simulink model "FOC_physical_2"  (R2024b)
settings: Solver=FixedStepAuto  StartTime=0.0  StopTime=3  FixedStep=1e-5  RelTol=1e-3
undefined symbols (not defined in the file): Down, GPTRIP1SEL, Ki_current, Ki_q, Ki_s, Ki_speed, Kp_current, Kp_q, Kp_s, Kp_speed, lambda, lamdaM, Ld, Ls, ma, P, Rs, T_max, T_period, Ts, TZ1, Up, Vdc
libraries: simulink x8, spsIGBTDiodeLib x6, spsCurrentMeasurementLib x3, eeStairGenerator x3, nesl_utility x2, spsDCVoltageSourceLib x1, spsPermanentMagnetSynchronousMachineLib x1, c2802xlib x1, spsThreePhaseVIMeasurementLib x1, spsVoltageMeasurementLib x1, sps_lib x1
(part 1 of 2)
settings Model: Creator=ahmed  LastModifiedBy=ahmed
settings SolverCC: ZeroCrossAlgorithm=Adaptive
settings DebuggingCC: IgnoredZcDiagnostic=none

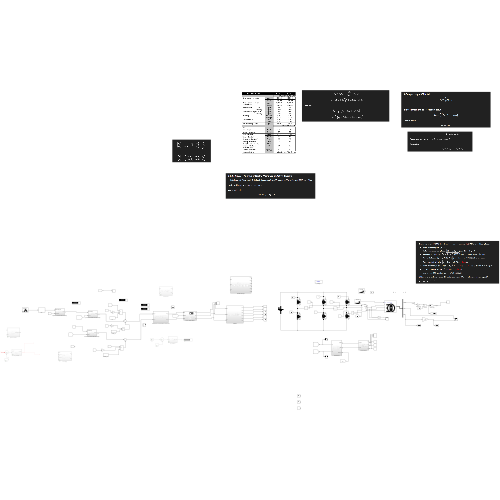
[thumbnail: Simulink's stored preview of the top-level diagram]
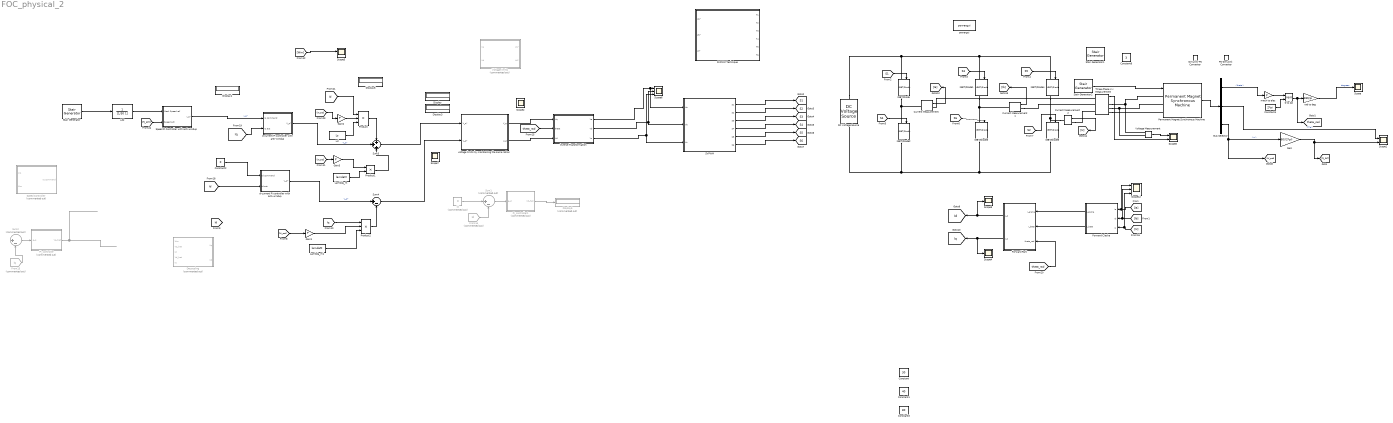
== system FOC_physical_2 ==
  0 to 2pi : Math  Operator=rem
  Bus Selector : BusSelector  OutputSignals=theta,Te,w
  Constant : Constant  Value=30
  Constant1 : Constant  Value=40
  Constant2 : Constant  Value=0
  Constant3 : Constant  Value=80
  Constant4 : Constant  Value=2*pi
  Constant6 : Constant  Value=3
  Current Measurement : spsCurrentMeasurementLib/Current Measurement  PhasorSimulation=off  OutputType=Complex  PSBequivalent=0
  Current Measurement1 : spsCurrentMeasurementLib/Current Measurement  PhasorSimulation=off  OutputType=Complex  PSBequivalent=0
  Current Measurement2 : spsCurrentMeasurementLib/Current Measurement  PhasorSimulation=off  OutputType=Complex  PSBequivalent=0
  DC Voltage Source : spsDCVoltageSourceLib/DC Voltage Source  Amplitude=Vdc  Measurements=None
  "Decoupling " : Subsystem  Commented=on
  Display{,3..4,6} (4 alike) : Display
  Display5 : Display  Commented=on
  Forward Clacke : Subsystem
  Forward Park : Subsystem
  From13 : From  Commented=on  GotoTag=Iq  TagVisibility=global
  From14 : From  Commented=on  GotoTag=Id  TagVisibility=global
  Gain : Gain  Gain=60/(2*pi)
  Gain1 : Gain  Gain=P
  Gain2 : Gain  Gain=P
  Gain3 : Gain  Gain=P
  IGBT/Diode{,1..5} (6 alike) : spsIGBTDiodeLib/IGBT//Diode  Ron=1e-3  Rs=1e5  Cs=inf  Measurements=on
  Id : Constant  Commented=on  Value=0
  Inverse Transformation : Subsystem
  LPF : TransferFcn  Denominator=[1/30 1]
  Lambda_m : Constant  Value=lamdaM
  Lambda_m1 : Constant  Value=lamdaM
  Ld : Constant  Value=Ls
  PI_controller : Subsystem  Commented=on
  PI_controller1 : Subsystem  Commented=on
  PS-Simulink Converter : nesl_utility/PS-Simulink Converter  PhysicalDomain=network_engine_domain  SubClassName=ps_output  LeftPortType=input  RightPortType=output  PseudoPeriodic=off  Frequencies=[]  VectorFormat=inherit  Unit=inherit  AffineConversion=off
  Permanent Magnet Synchronous Machine : spsPermanentMagnetSynchronousMachineLib/Permanent Magnet Synchronous Machine  NbPhases=3  FluxDistribution=Sinusoidal  RotorType=Round  MechanicalLoad=Torque Tm  PresetModel=No  ShowDetailedParameters=on  MeasurementBus=on  Resistance=Rs  Inductance=8.5e-3  dqInductances=[6.2e-3 6.2e-3]  La=Ls  MachineConstant=Flux linkage established by magnets (V.s)  Flux=.0620  VoltageCst=44.9822  TorqueCst=0.372  Flat=120  Mechanical=[2.6e-5 9.55e-5 4 .03]  PolePairs=4  InitialConditions=[0,0, 0,0]  InitialConditions5ph=[0 0 0 0 0 0]  RefAngle=Aligned with phase A axis (original Park)  IterativeDiscreteModel=Trapezoidal non iterative  TsBlock=-1  TsPowergui=0
  Product : Product  Inputs=3
  Product1 : Product
  Product2 : Product  Inputs=3
  SVPWM : Subsystem
  SVPWM Technique : Subsystem
  Scope : Scope
  Scope1 : Scope  NumInputPorts=2
  Scope{2,6..7,12} (4 alike) : Scope  NumInputPorts=3
  Scope3 : Scope
  Scope4 : Scope
  Scope5 : Scope  NumInputPorts=2
  Scope8 : Scope  NumInputPorts=2
  Simulink-PS Converter : nesl_utility/Simulink-PS Converter  PhysicalDomain=network_engine_domain  SubClassName=ps_input  LeftPortType=input  RightPortType=output  PseudoPeriodic=off  Frequencies=[]  NoiseDistribution=none  NoiseParameters=[]  Unit=1  AffineConversion=off  FilteringAndDerivatives=provide  SimscapeFilterOrder=1  InputFilterTimeConstant=0.001  UdotUserProvided=0
  "Speed Controller " : Subsystem  Commented=on
  Speed PI Controller with anti-windup : Subsystem
  Stair Generator : eeStairGenerator/Stair Generator  LabelModeActiveChoice=Discrete  TimeInput=[0.2 .6 1 1.3 1.8 2.2 3]  AmplitudeInput=[200 300 1000 4000 4500 2000 0]  SampleTime=1e-5  RepeatPattern=off  OutDataTypeStr=double
      settings: LibrarySourceBlock=ee_sl_lib/General Control/Stair Generator
  Stair Generator1 : eeStairGenerator/Stair Generator  LabelModeActiveChoice=Discrete  TimeInput=[0.3 .6 1.2 1.8]  AmplitudeInput=[.5 1 1.2 3]  SampleTime=Ts  RepeatPattern=off  OutDataTypeStr=double
      settings: LibrarySourceBlock=ee_sl_lib/General Control/Stair Generator
  Stair Generator2 : eeStairGenerator/Stair Generator  LabelModeActiveChoice=Discrete  TimeInput=[0.3 .7]  AmplitudeInput=[.6 1]  SampleTime=1e-5  RepeatPattern=off  OutDataTypeStr=double
      settings: LibrarySourceBlock=ee_sl_lib/General Control/Stair Generator
  Sum1 : Sum  Commented=on  Inputs=|+-
  Sum2 : Sum  Commented=on  Inputs=|+-
  Sum3 : Sum  Inputs=+++
  Sum4 : Sum  Inputs=|+-
  Three-Phase V-I Measurement : spsThreePhaseVIMeasurementLib/Three-Phase V-I Measurement  VoltageMeasurement=phase-to-ground  SetLabelV=off  LabelV=Vabc  Vpu=off  VpuLL=off  CurrentMeasurement=yes  SetLabelI=off  LabelI=Iabc  Ipu=off  Pbase=100e6  Vbase=500e3  OutputType=Complex  PhasorSimulation=off  PSBequivalent=0
  Voltage Measurement : spsVoltageMeasurementLib/Voltage Measurement  PhasorSimulation=off  OutputType=Complex  PSBequivalent=0
  Voltage limits : Subsystem  Commented=on
  d-current PI controller with anti-windup : Subsystem
  mech to elec : Gain  Gain=P
  powergui : sps_lib/powergui  Priority=1  SimulationMode=Discrete  SampleTime=1e-5  frequency=60  Iterations=50  frequencyindice=0  Pbase=100e6  ErrMax=1e-4  UnitsV=kV  UnitsW=MW  buscounter=0  FunctionMessages=off  echomessages=off  EnableUseOfTLC=off  CurrentSourceSwitches=off  DisableSnubberDevices=off  DisableRonSwitches=off  DisableVfSwitches=off  DisplayEquations=off  AutomaticDiscreteSolvers=off  SolverType=Tustin/Backward Euler (TBE)  Interpol=off  ExternalGateDelay=off  methode=off  Ts=100  x0status=blocks  SPID=on  SwTol=0  HookPort=off  NonlinearTolerance=1e-4  nMaxIteration=100  ContinueOnMaxIteration=off  RestoreLinks=warning  ResistiveCurrentMeasurement=off  Frange=[0:2:500]  Ylog=off  Xlog=on  ShowGrid=off  save=off  variable=ZData  structure=0  ZoomFFT=off  StartTime=0.0  cycles=1  DisplayStyle=1  fundamental=60  FreqAxis=off  MaxFrequency=1000  frequencyindicesteady=1  RmsSteady=1  display=off
  q-current PI controller with anti-windup : Subsystem
  rad to deg : Gain  Gain=180/pi
  voltage limits by maintaining the same ration : Subsystem
  tag scope: Id=global, Iq=global, S1=global, S2=global, S3=global, S4=global, S5=global, S6=global, theta_rad=global
  wires:
  Permanent Magnet Synchronous Machine/1 -> Bus Selector/1
  [S3] -> IGBT/Diode1/1
  [S6] -> IGBT/Diode3/1
  [S5] -> IGBT/Diode4/1
  [S4] -> IGBT/Diode2/1
  [S1] -> IGBT/Diode/1
  [S2] -> IGBT/Diode5/1
  [Wm] -> Scope5/1
  PI_controller1/1(Vd_hat) -> Display5/1
  Id/1 -> Sum1/1
  Inverse Transformation/1(Va) -> SVPWM/1(Va), Scope6/1
  Inverse Transformation/3(Vc) -> SVPWM/3(Vc), Scope6/3
  [theta_rad] -> Inverse Transformation/2(theta)
  Inverse Transformation/2(Vb) -> SVPWM/2(Vb), Scope6/2
  From14/1 -> Sum1/2
  [Ic] -> Forward Clacke/3(Ic), Scope12/3
  [Ia] -> Forward Clacke/1(Ia), Scope12/1
  Forward Clacke/2(I_beta) -> Forward Park/2(I_beta)
  [Ib] -> Forward Clacke/2(Ib), Scope12/2
  Forward Clacke/1(I_alpha) -> Forward Park/1(I_alpha)
  Forward Park/1(I_d) -> [Id], Scope3/1
  Forward Park/2(I_q) -> [Iq], Scope4/1
  Current Measurement/1 -> [Ia]
  Current Measurement1/1 -> [Ib]
  voltage limits by maintaining the same ration/1(V_q) -> Inverse Transformation/1(Vq)
  voltage limits by maintaining the same ration/2(V_d) -> Inverse Transformation/3(Vd)
  Sum1/1 -> PI_controller1/1(e_d)
  Constant2/1 -> d-current PI controller with anti-windup/1(Id command)
  [Id] -> d-current PI controller with anti-windup/2(Id act)
  ? -> Sum2/1
  Sum2/1 -> PI_controller/1(e_q)
  PI_controller/1(Vq_hat) -> ?
  From13/1 -> Sum2/2
  [Iq] -> q-current PI controller with anti-windup/2(Iq act)
  LPF/1 -> Speed PI Controller with anti-windup/1(Mech Speed ref)
  Speed PI Controller with anti-windup/1(I_q*) -> q-current PI controller with anti-windup/1(Iq command)  "I_q*"
  Product/1 -> Sum3/1
  [Iq] -> Product2/1
  Product1/1 -> Sum3/3
  Lambda_m1/1 -> Product2/3
  Lambda_m/1 -> Product1/2
  Ld/1 -> Product/3
  [W_act] -> Gain3/1
  Product2/1 -> Sum4/2
  [Id] -> Product/1
  q-current PI controller with anti-windup/1(V_q*) -> Sum3/2  "V_q*"
  Sum3/1 -> voltage limits by maintaining the same ration/1(V_q*)
  d-current PI controller with anti-windup/1(V_d*) -> Sum4/1  "V_d*"
  Sum4/1 -> voltage limits by maintaining the same ration/2(V_d*)
  Bus Selector/2 -> Scope1/1  "<Te>"
  Bus Selector/3 -> Gain/1, [W_act]  "<w>"
  Bus Selector/1 -> mech to elec/1  "<theta>"
  0 to 2pi/1 -> rad to deg/1, [theta_rad]
  Constant4/1 -> 0 to 2pi/2
  rad to deg/1 -> Scope/1  "degrees"
  mech to elec/1 -> 0 to 2pi/1
  Gain/1 -> Scope1/2, [N_act]
  [N_act] -> Speed PI Controller with anti-windup/2(Speed act)
  [W_act] -> Gain1/1
  [theta_rad] -> Forward Park/3(theta_rad)
  Current Measurement2/1 -> [Ic]
  Gain1/1 -> Product2/2
  [W_act] -> Gain2/1
  Gain2/1 -> Product/2
  SVPWM/1(S1) -> [S1]
  SVPWM/2(S2) -> [S2]
  SVPWM/3(S3) -> [S3]
  SVPWM/4(S4) -> [S4]
  SVPWM/5(S5) -> [S5]
  SVPWM/6(S6) -> [S6]
  Stair Generator/1 -> LPF/1
  Stair Generator2/1 -> Permanent Magnet Synchronous Machine/1
  Gain3/1 -> Product1/1
  Voltage Measurement/1 -> Scope8/1
  Three-Phase V-I Measurement/1 -> Scope8/2
  connections:
  DC Voltage Source/RConn1 -- IGBT/Diode4/LConn1 -- IGBT/Diode1/LConn1 -- IGBT/Diode/LConn1
  Current Measurement/LConn1 -- IGBT/Diode/RConn1 -- IGBT/Diode2/LConn1
  Current Measurement2/LConn1 -- IGBT/Diode4/RConn1 -- IGBT/Diode5/LConn1
  DC Voltage Source/LConn1 -- IGBT/Diode5/RConn1 -- IGBT/Diode3/RConn1 -- IGBT/Diode2/RConn1
  Current Measurement1/LConn1 -- IGBT/Diode1/RConn1 -- IGBT/Diode3/LConn1
  Voltage Measurement/LConn1 -- Permanent Magnet Synchronous Machine/LConn1 -- Three-Phase V-I Measurement/RConn1
  Voltage Measurement/LConn2 -- Permanent Magnet Synchronous Machine/LConn2 -- Three-Phase V-I Measurement/RConn2
  Current Measurement2/RConn1 -- Three-Phase V-I Measurement/LConn3
  Current Measurement1/RConn1 -- Three-Phase V-I Measurement/LConn2
  Three-Phase V-I Measurement/LConn1 -- Current Measurement/RConn1
  Three-Phase V-I Measurement/RConn3 -- Permanent Magnet Synchronous Machine/LConn3

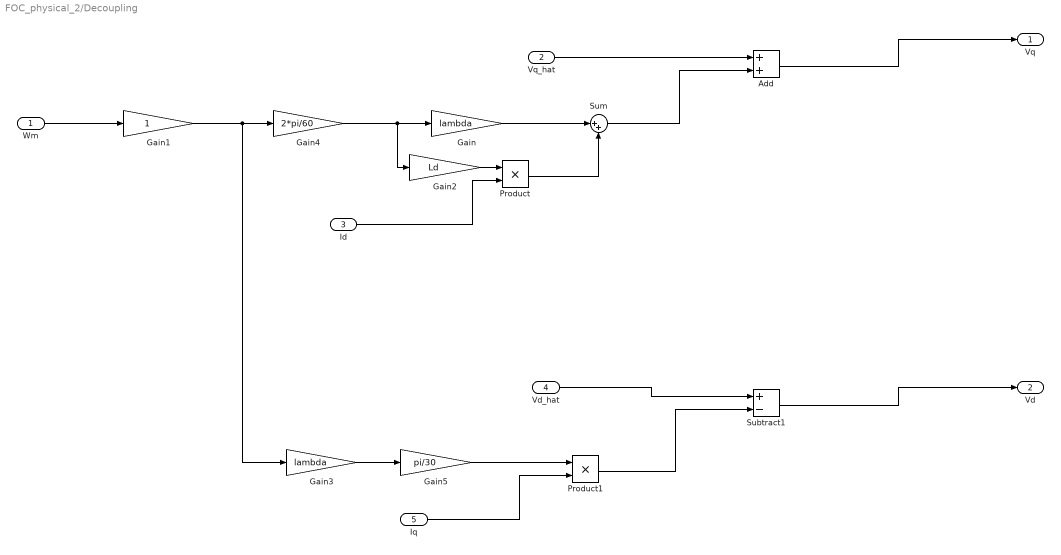
== system FOC_physical_2/Decoupling  ==
  Wm : Inport
  Vq_hat : Inport  Port=2
  Id : Inport  Port=3
  Vd_hat : Inport  Port=4
  Iq : Inport  Port=5
  Add : Sum
  Gain : Gain  Gain=lambda
  Gain1 : Gain
  Gain2 : Gain  Gain=Ld
  Gain3 : Gain  Gain=lambda
  Gain4 : Gain  Gain=2*pi/60
  Gain5 : Gain  Gain=pi/30
  Product : Product
  Product1 : Product
  Subtract1 : Sum  Inputs=+-
  Sum : Sum  Inputs=|++
  Vq : Outport
  Vd : Outport  Port=2
  wires:
  Vq_hat/1 -> Add/1
  Vd_hat/1 -> Subtract1/1
  Wm/1 -> Gain1/1
  Gain1/1 -> Gain4/1, Gain3/1
  Gain2/1 -> Product/1
  Id/1 -> Product/2
  Product/1 -> Sum/2
  Gain/1 -> Sum/1
  Sum/1 -> Add/2
  Gain3/1 -> Gain5/1
  Product1/1 -> Subtract1/2
  Iq/1 -> Product1/2
  Gain4/1 -> Gain2/1, Gain/1
  Add/1 -> Vq/1
  Subtract1/1 -> Vd/1
  Gain5/1 -> Product1/1

== system FOC_physical_2/Forward Clacke ==
  Ia : Inport
  Ib : Inport  Port=2
  Ic : Inport  Port=3
  Gain : Gain  Gain=0.5
  Gain1 : Gain  Gain=0.5
  Gain2 : Gain  Gain=2/3
  Gain3 : Gain  Gain=sqrt(3)/2
  Gain4 : Gain  Gain=2/3
  Sum : Sum  Inputs=+--
  Sum1 : Sum  Inputs=+-
  I_alpha : Outport
  I_beta : Outport  Port=2
  wires:
  Ib/1 -> Gain/1, Sum1/1
  Gain/1 -> Sum/2
  Gain2/1 -> I_alpha/1
  Sum1/1 -> Gain3/1
  Gain1/1 -> Sum/3
  Ic/1 -> Gain1/1, Sum1/2
  Sum/1 -> Gain2/1
  Gain3/1 -> Gain4/1
  Ia/1 -> Sum/1
  Gain4/1 -> I_beta/1

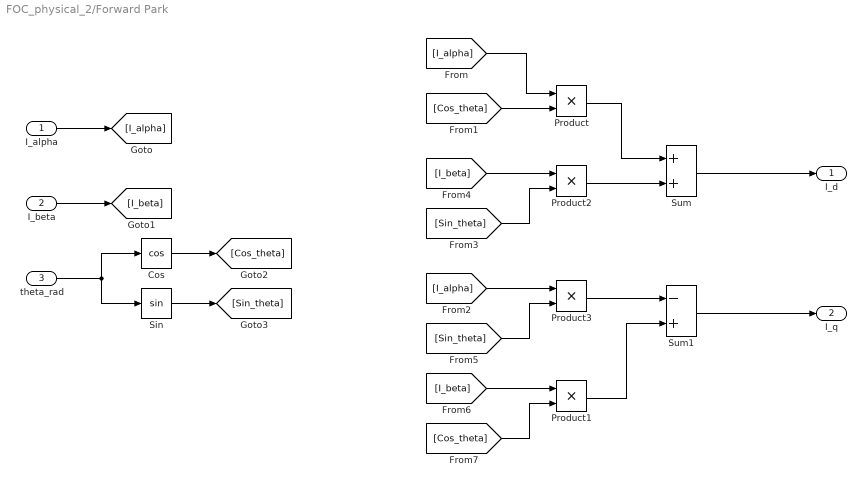
== system FOC_physical_2/Forward Park ==
  I_alpha : Inport
  I_beta : Inport  Port=2
  theta_rad : Inport  Port=3
  Cos : Trigonometry  Operator=cos
  Product{,1..3} (4 alike) : Product
  Sin : Trigonometry
  Sum : Sum
  Sum1 : Sum  Inputs=-+
  I_d : Outport
  I_q : Outport  Port=2
  wires:
  [Cos_theta] -> Product1/2
  [I_beta] -> Product1/1
  [Sin_theta] -> Product3/2
  [I_alpha] -> Product3/1
  Product1/1 -> Sum1/2
  [I_beta] -> Product2/1
  [Sin_theta] -> Product2/2
  [Cos_theta] -> Product/2
  Sin/1 -> [Sin_theta]
  Cos/1 -> [Cos_theta]
  theta_rad/1 -> Cos/1, Sin/1
  [I_alpha] -> Product/1
  I_beta/1 -> [I_beta]
  I_alpha/1 -> [I_alpha]
  Product3/1 -> Sum1/1
  Product2/1 -> Sum/2
  Product/1 -> Sum/1
  Sum1/1 -> I_q/1
  Sum/1 -> I_d/1

== system FOC_physical_2/Inverse Transformation ==
  Vq : Inport
  theta : Inport  Port=2
  Vd : Inport  Port=3
  "Inverse Park " : Subsystem  Commented=on
  dq to abc : Subsystem
  inverse Clark : Subsystem  Commented=on
  Va : Outport
  Vb : Outport  Port=2
  Vc : Outport  Port=3
  wires:
  theta/1 -> dq to abc/3(theta)
  Vq/1 -> dq to abc/1(V_q*)
  Vd/1 -> dq to abc/2(V_d*)
  dq to abc/1(Va*) -> Va/1
  dq to abc/2(Vb*) -> Vb/1
  dq to abc/3(Vc*) -> Vc/1

== system FOC_physical_2/PI_controller ==
  note: Kp = ((2*zeta*wn)-(Rs/ld))*Ld
  note: Kp = (Wn^2)*Ld
  e_q : Inport
  Add : Sum
  Display : Display
  Integrator : Integrator
  Ki : Gain  Gain=Ki_q
  Kp : Gain  Gain=Kp_q
  Product : Product
  Scope : Scope
  Vq_hat : Outport
  wires:
  Kp/1 -> Add/1
  Add/1 -> Vq_hat/1, Display/1
  e_q/1 -> Ki/1, Kp/1
  [Stop_q_integrator] -> Scope/1, Product/2
  Product/1 -> Integrator/1
  Integrator/1 -> Add/2
  Ki/1 -> Product/1

== system FOC_physical_2/PI_controller1 ==
  e_d : Inport
  Integrator : Integrator
  Ki : Gain  Gain=Ki_q
  Kp : Gain  Gain=Kp_q
  Product : Product
  Sum : Sum  Inputs=|++
  Time Scope : Scope
  Vd_hat : Outport
  wires:
  Kp/1 -> Sum/1
  e_d/1 -> Ki/1, Kp/1
  Sum/1 -> Vd_hat/1
  Product/1 -> Integrator/1
  [Stop_d_integrator] -> Product/2, Time Scope/1
  Integrator/1 -> Sum/2
  Ki/1 -> Product/1

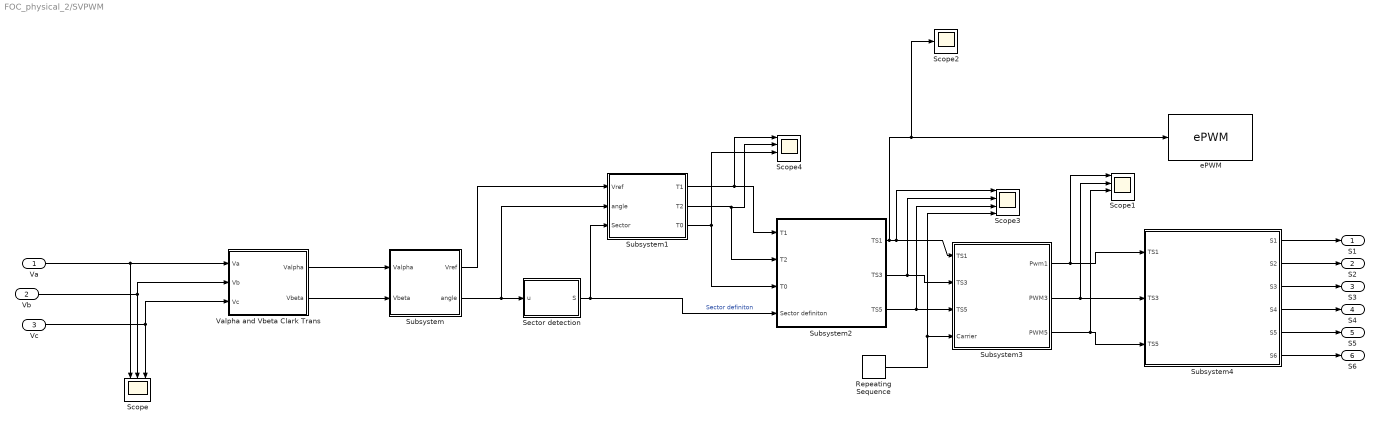
== system FOC_physical_2/SVPWM ==
  Va : Inport
  Vb : Inport  Port=2
  Vc : Inport  Port=3
  Repeating Sequence : simulink/Sources/Repeating Sequence  rep_seq_t="[0 (T_period)/2  (T_period) ]"  rep_seq_y=[0 (T_period) 0]
  Scope : Scope  NumInputPorts=3
  Scope1 : Scope  NumInputPorts=4
  Scope2 : Scope
  Scope3 : Scope  NumInputPorts=4
  Scope4 : Scope  NumInputPorts=4
  Sector detection : MATLAB Function  TreatAsAtomicUnit=on
  Subsystem : Subsystem
  Subsystem1 : Subsystem
  Subsystem2 : Subsystem
  Subsystem3 : Subsystem
  Subsystem4 : Subsystem
  Valpha and Vbeta Clark Trans : Subsystem
  ePWM : c2802xlib/ePWM  PwmType=C2000_Type4  useModule=ePWM1  ePWMxLINKTBPRD=Not Linked  periodUnits=Clock cycles  timerSource=Specify via dialog  timerPeriod_clk=64000  timerPeriod_sec=0.0001  tbshadow=Counter equals to zero  countingMode=Up-Down  phaseActiveEnable=Disable  phaseDirection=Count down after sync  phaseActive=0  synchronizationEnable=off  dcaevt1Sync=off  dcbevt1Sync=off  synchronizationOption=Disable  dcbevt1SyncOut=off  dcaevt1SyncOut=off  cmpdSyncOut=off  cmpcSyncOut=off  cmpbSyncOut=off  zeroSyncOut=off  swfSyncOut=off  perSynchronizationOption=Counter equals to period (CTR=PRD)  clockPrescale=1  HSclockPrescale=1  enswap=off  ePWMxAStatus=on  ePWMxAactionLogic1=Do nothing  ePWMxAactionLogic2=Do nothing  ePWMxAactionLogic3=Clear  ePWMxAactionLogic4=Set  ePWMxAactionLogic5=Do nothing  ePWMxAactionLogic6=Do nothing  ePWMxACSFenable=off  ePWMxACSFvalue=Forcing disable  ePWMxASFreload=Zero  ePWMxBStatus=on  ePWMxBactionLogic1=Do nothing  ePWMxBactionLogic2=Do nothing  ePWMxBactionLogic3=Set  ePWMxBactionLogic4=Clear  ePWMxBactionLogic5=Do nothing  ePWMxBactionLogic6=Do nothing  ePWMxBCSFenable=off  ePWMxBCSFvalue=Forcing disable  ePWMxBSFreload=Zero  ePWNxBOutWay=off  ePWMxLINKCMPA=Not Linked  CMPAUnits=Percentages  CMPASource=Input port  CMPAValue_per=0  CMPAValue_clk=32000  enCMPAshadow=Counter equals to zero (CTR=Zero)  ePWMxLINKCMPB=Not Linked  CMPBUnits=Clock cycles  CMPBSource=Specify via dialog  CMPBValue_per=50  CMPBValue_clk=32000  enCMPBshadow=Counter equals to zero (CTR=Zero)  ePWMxLINKCMPC=Not Linked  CMPCUnits=Clock cycles  CMPCSource=Specify via dialog  CMPCValue_per=50  CMPCValue_clk=32000  enCMPCshadow=Counter equals to zero (CTR=Zero)  ePWMxLINKCMPD=Not Linked  CMPDUnits=Clock cycles  CMPDSource=Specify via dialog  CMPDValue_per=50  CMPDValue_clk=32000  enCMPDshadow=Counter equals to zero (CTR=Zero)  enableDBePWMxA=on  enableDBePWMxB=on  enhalfcycle=off  DBpolarity=Active high complementary (AHC)  DBedgeDelay=Positive  DBSource_ePWMxA=ePWMxA  DBSource_ePWMxB=ePWMxA  DBPeriodUnits=Seconds  DBperiodSource=Specify via dialog  REDperiod=0  FEDperiod=0  REDperiod_sec=1e-6  FEDperiod_sec=1e-6  LoadModeDBRED=Immediate without using shadow  LoadModeDBFED=Immediate without using shadow  adcstartModuleA=off  adcrequestEventA=First event  adcstartEventA=Digital Compare Module A Event 1 start of conversion (DCAEVT1.soc)  adcstartEventA_type2=Counter equals to zero (CTR=Zero)  adcstartModuleB=off  adcrequestEventB=First event  adcstartEventB=Counter equals to zero (CTR=Zero)  adcstartEventB_type2=Counter equals to zero (CTR=Zero)  intEn=off  intPrd=First event  intSel=Counter equals to zero (CTR=Zero)  intSel_type2=Counter equals to zero (CTR=Zero)  hrpe=off  enHRPWM=off  HRPWM_LoadMode=Counter equals to period (CTR=PRD)  HRPWM_CTLMode=Duty or Period control mode  HRPWM_EDGMode=Both edge  hrpeb=off  enHRPWMB=off  HRPWM_LoadModeB=Counter equals to zero (CTR=ZERO)  HRPWM_CTLModeB=Duty or Period control mode  HRPWM_EDGModeB=Both edge  enHRDBRED=off  enHRDBFED=off  enSFO=on  enautoconv=on  chopperEnable=off  chopperFrequency=1  chopperFirstwidth=1  chopperDuty=12.5%  tripZonesource=Specify via dialog  tzselOSHT1=off  tzselOSHT2=off  tzselOSHT3=off  tzselOSHT4=off  tzselOSHT5=off  tzselOSHT6=off  tzselOSHDCAEV1=off  tzselOSHDCBEV1=off  tzselCBC1=off  tzselCBC2=off  tzselCBC3=off  tzselCBC4=off  tzselCBC5=off  tzselCBC6=off  tzselCBCDCAEV2=off  tzselCBCDCBEV2=off  enTzOstIntr=off  enTzCbcIntr=off  enTzDCAEVT1Intr=off  enTzDCAEVT2Intr=off  enTzDCBEVT1Intr=off  enTzDCBEVT2Intr=off  tzclrCBCLatch=Counter equals to zero (CTR=Zero)  ePWMxAforced=No action  ePWMxBforced=No action  DCAEVT1forced=No action  DCBEVT1forced=No action  DCAEVT2forced=No action  DCBEVT2forced=No action  dcah=Trip Zone 1 input (TZ1)  dcal=Trip Zone 2 input (TZ2)  dcbh=Trip Zone 1 input (TZ1)  dcbl=Trip Zone 2 input (TZ2)  dcah_type2=GPTRIP1SEL/(TZ1)  dcal_type2=GPTRIP1SEL/(TZ1)  dcbh_type2=GPTRIP1SEL/(TZ1)  dcbl_type2=GPTRIP1SEL/(TZ1)  gendcaevt1=Event disabled  gendcaevt2=Event disabled  gendcbevt1=Event disabled  gendcbevt2=Event disabled  dcaevt1src=DCAEVT1 with sync  dcaevt2src=DCAEVT2 with sync  dcbevt1src=DCBEVT1 with sync  dcbevt2src=DCBEVT2 with sync  pulsesel=Counter equals to zero (CTR=Zero)  blankinv=off  blankoffset=0  blankwidth=0  evsrcsel=Filtered version of DCAEVT1 (DCAEVT1FILT)  encape=off
  S1 : Outport
  S2 : Outport  Port=2
  S3 : Outport  Port=3
  S4 : Outport  Port=4
  S5 : Outport  Port=5
  S6 : Outport  Port=6
  wires:
  Subsystem4/5(S5) -> S5/1
  Sector detection/1(S) -> Subsystem2/4(Sector definiton), Subsystem1/3(Sector)  "Sector definiton"
  Subsystem/2(angle) -> Sector detection/1(u), Subsystem1/2(angle)
  Subsystem/1(Vref) -> Subsystem1/1(Vref)
  Valpha and Vbeta Clark Trans/2(Vbeta) -> Subsystem/2(Vbeta)
  Va/1 -> Valpha and Vbeta Clark Trans/1(Va), Scope/1
  Repeating Sequence/1 -> Scope3/4, Subsystem3/4(Carrier)
  Valpha and Vbeta Clark Trans/1(Valpha) -> Subsystem/1(Valpha)
  Vb/1 -> Valpha and Vbeta Clark Trans/2(Vb), Scope/2
  Vc/1 -> Valpha and Vbeta Clark Trans/3(Vc), Scope/3
  Subsystem1/2(T2) -> Scope4/2, Subsystem2/2(T2)
  Subsystem1/1(T1) -> Scope4/1, Subsystem2/1(T1)
  Subsystem1/3(T0) -> Subsystem2/3(T0), Scope4/3
  Subsystem2/1(TS1) -> Scope2/1, ePWM/1, Subsystem3/1(TS1), Scope3/1
  Subsystem2/2(TS3) -> Subsystem3/2(TS3), Scope3/2
  Subsystem2/3(TS5) -> Subsystem3/3(TS5), Scope3/3
  Subsystem3/1(Pwm1) -> Scope1/1, Subsystem4/1(TS1)
  Subsystem3/2(PWM3) -> Scope1/2, Subsystem4/2(TS3)
  Subsystem3/3(PWM5) -> Scope1/3, Subsystem4/3(TS5)
  Subsystem4/1(S1) -> S1/1
  Subsystem4/2(S2) -> S2/1
  Subsystem4/3(S3) -> S3/1
  Subsystem4/4(S4) -> S4/1
  Subsystem4/6(S6) -> S6/1

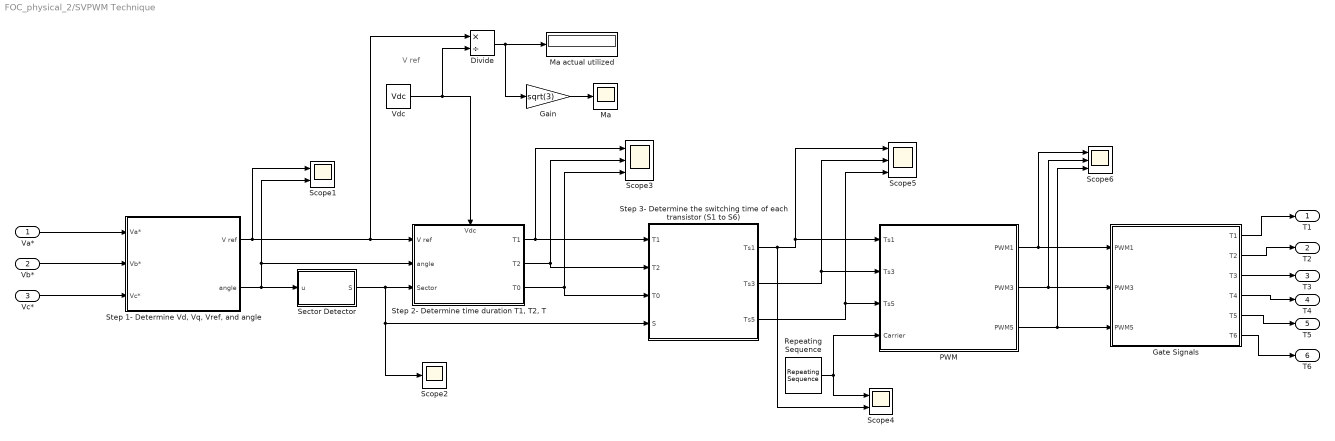
== system FOC_physical_2/SVPWM Technique ==
  note: V ref
  Va* : Inport
  Vb* : Inport  Port=2
  Vc* : Inport  Port=3
  Divide : Product  Inputs=*/
  Gain : Gain  Gain=sqrt(3)
  Gate Signals : Subsystem
  Ma : Scope
  Ma actual utilized : Display
  PWM : Subsystem
  Repeating Sequence : simulink/Sources/Repeating Sequence  rep_seq_t=[ 0 (T_period)/2 (T_period) ]  rep_seq_y=[ 0 (T_period) 0 ]
  Scope1 : Scope  NumInputPorts=2
  Scope2 : Scope
  Scope3 : Scope  NumInputPorts=3
  Scope4 : Scope  NumInputPorts=2
  Scope5 : Scope  NumInputPorts=3
  Scope6 : Scope  NumInputPorts=3
  Sector Detector : MATLAB Function  TreatAsAtomicUnit=on
  "Step 1- Determine Vd, Vq, Vref, and angle" : Subsystem
  "Step 2- Determine time duration T1, T2, T" : Subsystem
      settings: PortSchema="{\"entries\":[{\"content\":{\"sides\":[{\"content\":{\"connectorIds\":[\"In1\",\"In2\",\"In3\"]},\"type\":\"ConnectorPlacement.EquallySpacedRectSide\",\"uuid\":\"2dad9b71-fb55-40e3-9250-08671b06fd76\"},{\"content\":{\"connectorIds\":[\"Out1\",\"Out2\",\"Out3\"],\"side\":\"RIGHT\"},\"type\":\"ConnectorPlacement.EquallySpacedRectSide\",\"uuid\":\"fd9577f6-2035-4946-b366-efd909fd578d\"},{\"content\":{\"connectorIds\":[\"In4\"],\"side\":\"TOP\"},\"type\":\"ConnectorPlacement.EquallySpacedRectSide\",\"uuid\":\"03f93542-188d-4be0-9359-187a882052ac\"}]},\"type\":\"ConnectorPlacement.EquallySpacedConnector\",\"uuid\":\"0cec5607-3333-48e6-b527-ee7f13af7673\"}],\"packageUris\":[\"http://schema.mathworks.com/mf0/Connector/R2020b\"],\"version\":\"1.0\"}"
  "Step 3- Determine the switching time of each transistor (S1 to S6) " : Subsystem
  Vdc : Constant  Value=Vdc
  T1 : Outport
  T2 : Outport  Port=2
  T3 : Outport  Port=3
  T4 : Outport  Port=4
  T5 : Outport  Port=5
  T6 : Outport  Port=6
  wires:
  Vc*/1 -> "Step 1- Determine Vd, Vq, Vref, and angle"/3(Vc*)
  Vb*/1 -> "Step 1- Determine Vd, Vq, Vref, and angle"/2(Vb*)
  "Step 1- Determine Vd, Vq, Vref, and angle"/1(V ref) -> "Step 2- Determine time duration T1, T2, T"/1(V ref), Divide/1, Scope1/1
  Gate Signals/3(T3) -> T3/1
  Gate Signals/1(T1) -> T1/1
  Gate Signals/5(T5) -> T5/1
  "Step 3- Determine the switching time of each transistor (S1 to S6) "/3(Ts5) -> PWM/3(Ts5), Scope5/3
  "Step 3- Determine the switching time of each transistor (S1 to S6) "/2(Ts3) -> PWM/2(Ts3), Scope5/2
  "Step 3- Determine the switching time of each transistor (S1 to S6) "/1(Ts1) -> Scope4/2, PWM/1(Ts1), Scope5/1
  Gate Signals/6(T6) -> T6/1
  PWM/3(PWM5) -> Gate Signals/3(PWM5), Scope6/3
  Divide/1 -> Gain/1, Ma actual utilized/1
  Va*/1 -> "Step 1- Determine Vd, Vq, Vref, and angle"/1(Va*)
  "Step 2- Determine time duration T1, T2, T"/2(T2) -> "Step 3- Determine the switching time of each transistor (S1 to S6) "/2(T2), Scope3/2
  PWM/1(PWM1) -> Gate Signals/1(PWM1), Scope6/1
  "Step 2- Determine time duration T1, T2, T"/1(T1) -> "Step 3- Determine the switching time of each transistor (S1 to S6) "/1(T1), Scope3/1
  Gate Signals/2(T2) -> T2/1
  Vdc/1 -> "Step 2- Determine time duration T1, T2, T"/4(Vdc), Divide/2
  Sector Detector/1(S) -> Scope2/1, "Step 3- Determine the switching time of each transistor (S1 to S6) "/4(S), "Step 2- Determine time duration T1, T2, T"/3(Sector)
  Gate Signals/4(T4) -> T4/1
  PWM/2(PWM3) -> Gate Signals/2(PWM3), Scope6/2
  "Step 1- Determine Vd, Vq, Vref, and angle"/2(angle) -> Sector Detector/1(u), "Step 2- Determine time duration T1, T2, T"/2(angle), Scope1/2
  "Step 2- Determine time duration T1, T2, T"/3(T0) -> "Step 3- Determine the switching time of each transistor (S1 to S6) "/3(T0), Scope3/3
  Repeating Sequence/1 -> PWM/4(Carrier), Scope4/1
  Gain/1 -> Ma/1

== system FOC_physical_2/Speed Controller  ==
  In1 : Inport
  Wm : Inport  Port=2
  Abs : Abs  SaturateOnIntegerOverflow=off
  Abs1 : Abs  SaturateOnIntegerOverflow=off
  Add : Sum
  Compare To Constant : simulink/Logic and Bit Operations/Compare To Constant  relop=<=  const=.0001  OutDataTypeStr=boolean
  Display1 : Display
  Gain : Gain  Gain=Kp_s
  Gain1 : Gain  Gain=Ki_s
  Gain2 : Gain  Gain=2*pi/60
  Integrator : Integrator  ExternalReset=falling
  Product : Product  Inputs=3
  Relay : Relay  OnSwitchValue=100  OffSwitchValue=-100
  Saturation : Saturate  UpperLimit=11  LowerLimit=-11
  Sum : Sum  Inputs=|-+
  Sum1 : Sum  Inputs=|+-
  Iq command : Outport
  wires:
  Gain/1 -> Add/1
  Add/1 -> Saturation/1, Sum/2
  Gain2/1 -> Gain/1, Gain1/1
  In1/1 -> Sum1/1  "Wm"
  Wm/1 -> Abs/1, Sum1/2
  Sum1/1 -> Gain2/1
  Abs/1 -> Relay/1
  Product/1 -> Integrator/1
  Saturation/1 -> Sum/1, Iq command/1, Display1/1
  Abs1/1 -> Compare To Constant/1
  Sum/1 -> Abs1/1
  Compare To Constant/1 -> Product/1
  Gain1/1 -> Product/2
  Relay/1 -> Integrator/2, Product/3
  Integrator/1 -> Add/2

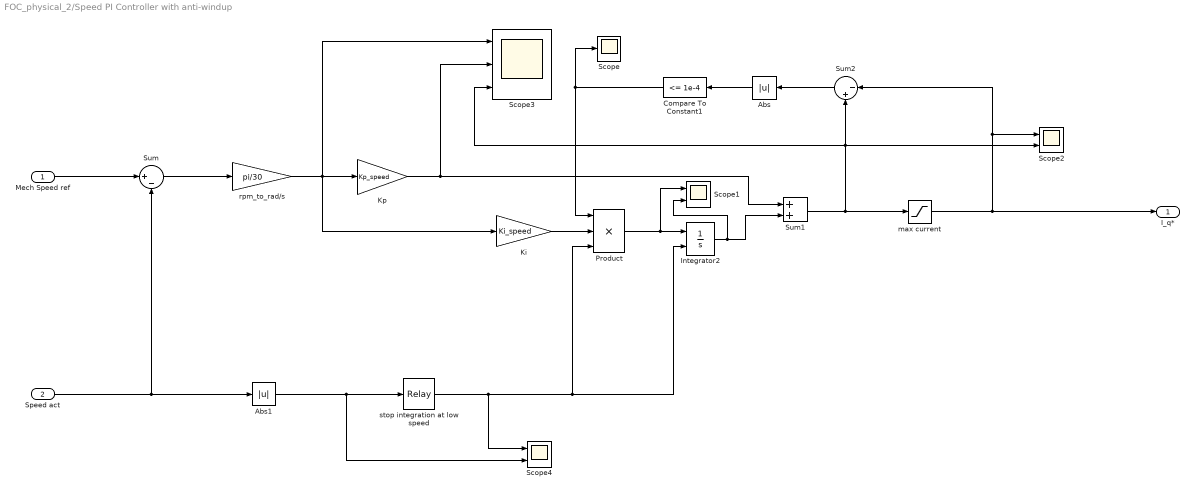
== system FOC_physical_2/Speed PI Controller with anti-windup ==
  Mech Speed ref : Inport
  Speed act : Inport  Port=2
  " max current" : Saturate  UpperLimit=T_max/((3/2)*lamdaM*P)  LowerLimit=0
  Abs : Abs  SaturateOnIntegerOverflow=off
  Abs1 : Abs  SaturateOnIntegerOverflow=off
  Compare To Constant1 : simulink/Logic and Bit Operations/Compare To Constant  relop=<=  const=1e-4  OutDataTypeStr=boolean
  Integrator2 : Integrator  ExternalReset=falling
  "Ki " : Gain  Gain=Ki_speed
  Kp : Gain  Gain=Kp_speed
  Product : Product  Inputs=3
  Scope : Scope
  Scope1 : Scope  NumInputPorts=2
  Scope2 : Scope  NumInputPorts=2
  Scope3 : Scope  NumInputPorts=3
  Scope4 : Scope  NumInputPorts=2
  Sum : Sum  Inputs=|+-
  Sum1 : Sum
  Sum2 : Sum  Inputs=|-+
  rpm_to_rad/s : Gain  Gain=pi/30
  stop integration at low speed : Relay  OnSwitchValue=100  OffSwitchValue=-100
  I_q* : Outport
  wires:
  " max current"/1 -> Scope2/1, Sum2/1, I_q*/1
  Sum/1 -> rpm_to_rad/s/1
  rpm_to_rad/s/1 -> Kp/1, Scope3/1, "Ki "/1
  stop integration at low speed/1 -> Integrator2/2, Product/3, Scope4/1
  Abs1/1 -> Scope4/2, stop integration at low speed/1
  Compare To Constant1/1 -> Scope/1, Product/1
  Abs/1 -> Compare To Constant1/1
  Sum2/1 -> Abs/1
  Sum1/1 -> " max current"/1, Sum2/2, Scope3/3, Scope2/2
  Integrator2/1 -> Sum1/2, Scope1/2
  Product/1 -> Integrator2/1, Scope1/1
  "Ki "/1 -> Product/2
  Kp/1 -> Sum1/1, Scope3/2
  Speed act/1 -> Sum/2, Abs1/1
  Mech Speed ref/1 -> Sum/1

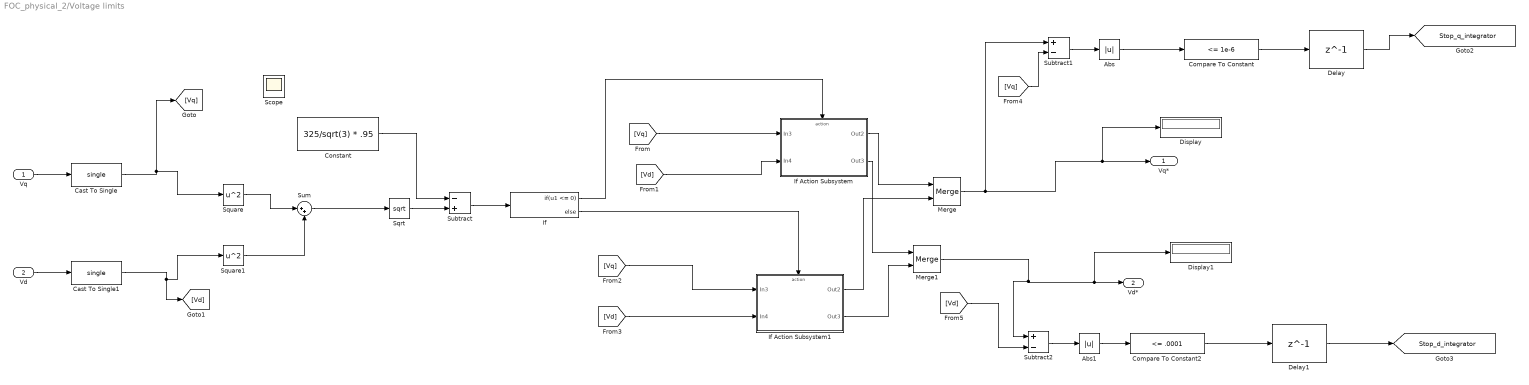
== system FOC_physical_2/Voltage limits ==
  Vq : Inport
  Vd : Inport  Port=2
  Abs : Abs  SaturateOnIntegerOverflow=off
  Abs1 : Abs  SaturateOnIntegerOverflow=off
  Cast To Single : DataTypeConversion  OutDataTypeStr=single  SaturateOnIntegerOverflow=off  RndMeth=Floor
  Cast To Single1 : DataTypeConversion  OutDataTypeStr=single  SaturateOnIntegerOverflow=off  RndMeth=Floor
  Compare To Constant : simulink/Logic and Bit Operations/Compare To Constant  relop=<=  const=1e-6  OutDataTypeStr=boolean
  Compare To Constant2 : simulink/Logic and Bit Operations/Compare To Constant  relop=<=  const=.0001  OutDataTypeStr=boolean
  Constant : Constant  Value=325/sqrt(3) * .95
  Delay : Delay  DelayLength=1
  Delay1 : Delay  DelayLength=1
  Display : Display
  Display1 : Display
  If : If  IfExpression=u1 <= 0
  If Action Subsystem : Subsystem  TreatAsAtomicUnit=on
  If Action Subsystem1 : Subsystem  TreatAsAtomicUnit=on
  Merge : Merge
  Merge1 : Merge
  Scope : Scope
  Sqrt : Sqrt
  Square : Math  Operator=square
  Square1 : Math  Operator=square
  Subtract : Sum  Inputs=-+
  Subtract1 : Sum  Inputs=+-
  Subtract2 : Sum  Inputs=+-
  Sum : Sum  Inputs=|++
  Vq* : Outport
  Vd* : Outport  Port=2
  tag scope: Stop_d_integrator=global, Stop_q_integrator=global
  wires:
  Vq/1 -> Cast To Single/1
  Vd/1 -> Cast To Single1/1
  Square/1 -> Sum/1
  Square1/1 -> Sum/2
  Sum/1 -> Sqrt/1
  Sqrt/1 -> Subtract/2
  Constant/1 -> Subtract/1
  Subtract/1 -> If/1
  If/1 -> If Action Subsystem/Action
  If/2 -> If Action Subsystem1/Action
  [Vq] -> If Action Subsystem/1(In3)
  [Vd] -> If Action Subsystem/2(In4)
  [Vq] -> If Action Subsystem1/1(In3)
  [Vd] -> If Action Subsystem1/2(In4)
  If Action Subsystem/1(Out2) -> Merge/1
  If Action Subsystem1/1(Out2) -> Merge/2
  If Action Subsystem/2(Out3) -> Merge1/1
  If Action Subsystem1/2(Out3) -> Merge1/2
  Merge/1 -> Subtract1/1, Display/1, Vq*/1
  Subtract1/1 -> Abs/1
  Abs/1 -> Compare To Constant/1
  Abs1/1 -> Compare To Constant2/1
  Subtract2/1 -> Abs1/1
  [Vd] -> Subtract2/2
  Compare To Constant/1 -> Delay/1
  Compare To Constant2/1 -> Delay1/1
  Delay/1 -> [Stop_q_integrator]
  Delay1/1 -> [Stop_d_integrator]
  Merge1/1 -> Subtract2/1, Display1/1, Vd*/1
  Cast To Single/1 -> [Vq], Square/1
  Cast To Single1/1 -> [Vd], Square1/1
  [Vq] -> Subtract1/2

== system FOC_physical_2/d-current PI controller with anti-windup ==
  Id command : Inport
  Id act : Inport  Port=2
  Integrator2 : Integrator
  "Ki " : Gain  Gain=Ki_current
  Kp : Gain  Gain=Kp_current
  Product : Product
  Scope : Scope
  Scope1 : Scope  NumInputPorts=2
  Scope2 : Scope  NumInputPorts=2
  Scope3 : Scope  NumInputPorts=3
  Sum : Sum  Inputs=|+-
  Sum1 : Sum
  V_d* : Outport
  wires:
  Sum1/1 -> V_d*/1, Scope3/3, Scope2/2
  Integrator2/1 -> Sum1/2, Scope1/2
  Product/1 -> Integrator2/1, Scope1/1
  "Ki "/1 -> Product/2
  Kp/1 -> Sum1/1, Scope3/2
  Sum/1 -> Kp/1, Scope3/1, "Ki "/1
  Id act/1 -> Sum/2
  Id command/1 -> Sum/1
  [stop_d_integrator] -> Product/1, Scope/1

== system FOC_physical_2/q-current PI controller with anti-windup ==
  Iq command : Inport
  Iq act : Inport  Port=2
  Integrator2 : Integrator
  "Ki " : Gain  Gain=Ki_current
  Kp : Gain  Gain=Kp_current
  Product : Product
  Scope : Scope
  Scope1 : Scope  NumInputPorts=2
  Scope2 : Scope  NumInputPorts=2
  Scope3 : Scope  NumInputPorts=3
  Sum : Sum  Inputs=|+-
  Sum1 : Sum
  V_q* : Outport
  wires:
  Iq command/1 -> Sum/1
  Iq act/1 -> Sum/2
  Sum/1 -> "Ki "/1, Scope3/1, Kp/1
  Kp/1 -> Scope3/2, Sum1/1
  "Ki "/1 -> Product/2
  Product/1 -> Integrator2/1, Scope1/1
  Integrator2/1 -> Scope1/2, Sum1/2
  Sum1/1 -> V_q*/1, Scope2/2, Scope3/3
  [stop_q_integrator] -> Scope/1, Product/1

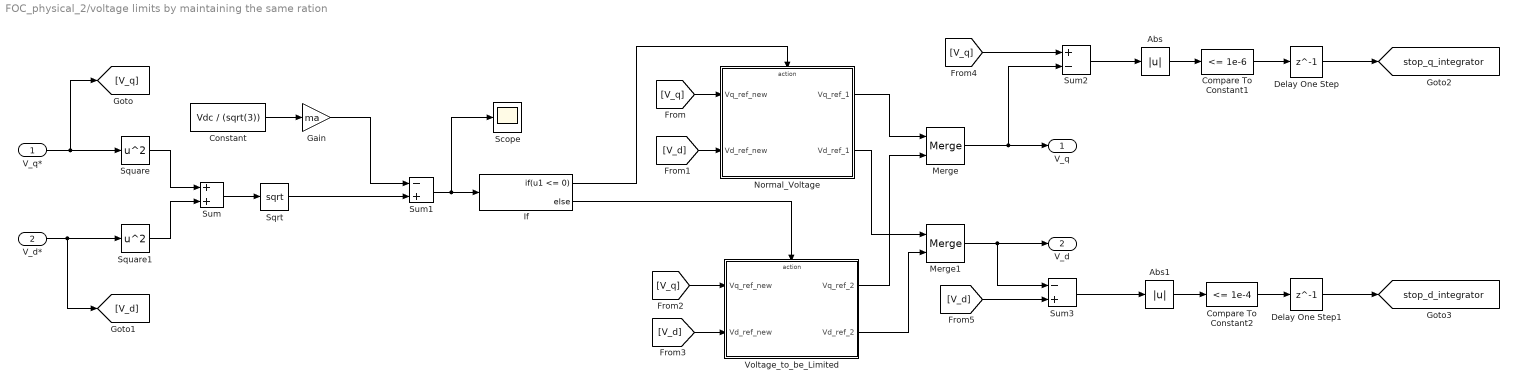
== system FOC_physical_2/voltage limits by maintaining the same ration ==
  V_q* : Inport
  V_d* : Inport  Port=2
  Abs : Abs  SaturateOnIntegerOverflow=off
  Abs1 : Abs  SaturateOnIntegerOverflow=off
  Compare To Constant1 : simulink/Logic and Bit Operations/Compare To Constant  relop=<=  const=1e-6  OutDataTypeStr=boolean
  Compare To Constant2 : simulink/Logic and Bit Operations/Compare To Constant  relop=<=  const=1e-4  OutDataTypeStr=boolean
  Constant : Constant  Value=Vdc / (sqrt(3))
  Delay One Step : Delay  DelayLength=1
  Delay One Step1 : Delay  DelayLength=1
  Gain : Gain  Gain=ma
  If : If  IfExpression=u1 <= 0
  Merge : Merge
  Merge1 : Merge
  Normal_Voltage : Subsystem  TreatAsAtomicUnit=on
      settings: RTWSystemCode=Inline  RTWFcnNameOpts=Use subsystem name  RTWFileNameOpts=Use subsystem name
  Scope : Scope
  Sqrt : Sqrt
  Square : Math  Operator=square
  Square1 : Math  Operator=square
  Sum : Sum
  Sum1 : Sum  Inputs=-+
  Sum2 : Sum  Inputs=+-
  Sum3 : Sum  Inputs=-+
  Voltage_to_be_Limited : Subsystem  TreatAsAtomicUnit=on
      settings: RTWSystemCode=Inline  RTWFcnNameOpts=Use subsystem name  RTWFileNameOpts=Use subsystem name
  V_q : Outport
  V_d : Outport  Port=2
  tag scope: stop_d_integrator=global, stop_q_integrator=global
  wires:
  V_q*/1 -> [V_q], Square/1
  V_d*/1 -> [V_d], Square1/1
  Sum/1 -> Sqrt/1
  Square/1 -> Sum/1
  Square1/1 -> Sum/2
  Sqrt/1 -> Sum1/2
  Merge/1 -> Sum2/2, V_q/1
  Constant/1 -> Gain/1
  Gain/1 -> Sum1/1
  Sum1/1 -> Scope/1, If/1
  If/1 -> Normal_Voltage/Action
  [V_q] -> Normal_Voltage/1(Vq_ref_new)
  [V_d] -> Normal_Voltage/2(Vd_ref_new)
  If/2 -> Voltage_to_be_Limited/Action
  Voltage_to_be_Limited/1(Vq_ref_2) -> Merge/2
  Normal_Voltage/1(Vq_ref_1) -> Merge/1
  Voltage_to_be_Limited/2(Vd_ref_2) -> Merge1/2
  Normal_Voltage/2(Vd_ref_1) -> Merge1/1
  [V_q] -> Voltage_to_be_Limited/1(Vq_ref_new)
  [V_d] -> Voltage_to_be_Limited/2(Vd_ref_new)
  [V_q] -> Sum2/1
  Merge1/1 -> Sum3/1, V_d/1
  [V_d] -> Sum3/2
  Delay One Step/1 -> [stop_q_integrator]
  Delay One Step1/1 -> [stop_d_integrator]
  Abs/1 -> Compare To Constant1/1
  Compare To Constant1/1 -> Delay One Step/1
  Sum2/1 -> Abs/1
  Sum3/1 -> Abs1/1
  Abs1/1 -> Compare To Constant2/1
  Compare To Constant2/1 -> Delay One Step1/1

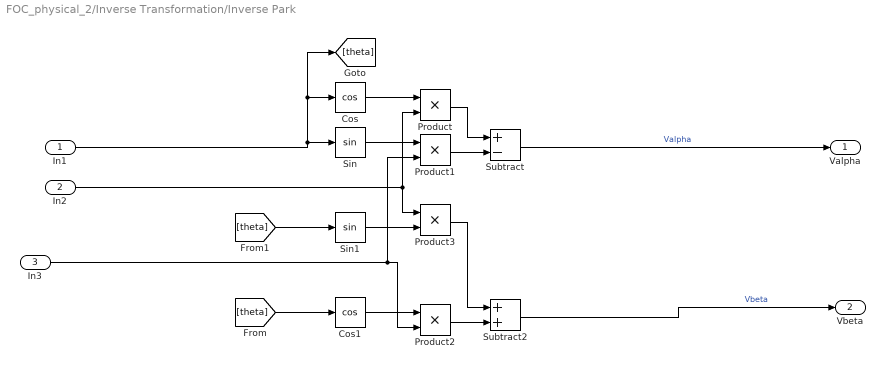
== system FOC_physical_2/Inverse Transformation/Inverse Park  ==
  In1 : Inport
  In2 : Inport  Port=2
  In3 : Inport  Port=3
  Cos : Trigonometry  Operator=cos
  Cos1 : Trigonometry  Operator=cos
  Product{,1..3} (4 alike) : Product
  Sin : Trigonometry
  Sin1 : Trigonometry
  Subtract : Sum  Inputs=+-
  Subtract2 : Sum
  Valpha : Outport
  Vbeta : Outport  Port=2
  wires:
  Product3/1 -> Subtract2/1
  In3/1 -> Product2/2, Product1/2
  In1/1 -> Cos/1, [theta], Sin/1
  Subtract/1 -> Valpha/1  "Valpha"
  Product/1 -> Subtract/1
  Subtract2/1 -> Vbeta/1  "Vbeta"
  Product2/1 -> Subtract2/2
  Cos/1 -> Product/1
  Product1/1 -> Subtract/2
  [theta] -> Cos1/1
  In2/1 -> Product/2, Product3/1
  [theta] -> Sin1/1
  Sin/1 -> Product1/1
  Cos1/1 -> Product2/1
  Sin1/1 -> Product3/2

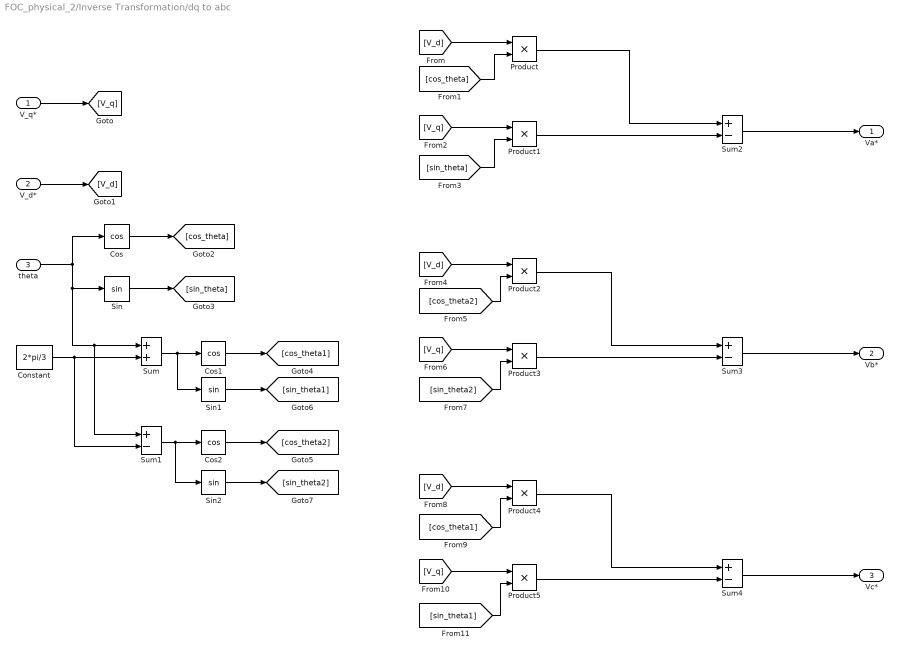
== system FOC_physical_2/Inverse Transformation/dq to abc ==
  V_q* : Inport
  V_d* : Inport  Port=2
  theta : Inport  Port=3
  Constant : Constant  Value=2*pi/3
  Cos : Trigonometry  Operator=cos
  Cos1 : Trigonometry  Operator=cos
  Cos2 : Trigonometry  Operator=cos
  Product{,1..5} (6 alike) : Product
  Sin : Trigonometry
  Sin1 : Trigonometry
  Sin2 : Trigonometry
  Sum : Sum
  Sum{1..4} (4 alike) : Sum  Inputs=+-
  Va* : Outport
  Vb* : Outport  Port=2
  Vc* : Outport  Port=3
  wires:
  [sin_theta1] -> Product5/2
  [V_q] -> Product5/1
  [cos_theta1] -> Product4/2
  [V_d] -> Product4/1
  Product4/1 -> Sum4/1
  Product5/1 -> Sum4/2
  Sum4/1 -> Vc*/1
  [sin_theta2] -> Product3/2
  Sin2/1 -> [sin_theta2]
  Sin1/1 -> [sin_theta1]
  [V_q] -> Product3/1
  [cos_theta2] -> Product2/2
  [V_d] -> Product2/1
  Sum3/1 -> Vb*/1
  Product3/1 -> Sum3/2
  Product2/1 -> Sum3/1
  [sin_theta] -> Product1/2
  [V_q] -> Product1/1
  [cos_theta] -> Product/2
  [V_d] -> Product/1
  Product/1 -> Sum2/1
  Product1/1 -> Sum2/2
  Sum2/1 -> Va*/1
  Cos2/1 -> [cos_theta2]
  Cos1/1 -> [cos_theta1]
  Sum1/1 -> Cos2/1, Sin2/1
  Sum/1 -> Cos1/1, Sin1/1
  Constant/1 -> Sum/2, Sum1/2
  Sin/1 -> [sin_theta]
  Cos/1 -> [cos_theta]
  theta/1 -> Cos/1, Sin/1, Sum1/1, Sum/1
  V_d*/1 -> [V_d]
  V_q*/1 -> [V_q]

== system FOC_physical_2/Inverse Transformation/inverse Clark ==
  In1 : Inport
  In2 : Inport  Port=2
  Add : Sum
  Add1 : Sum
  Constant : Constant  Value=-1/2
  Constant1 : Constant  Value=sqrt(3)/2
  Constant2 : Constant  Value=-1/2
  Constant3 : Constant  Value=-sqrt(3)/2
  Product{,1..3} (4 alike) : Product
  Va : Outport
  Vb : Outport  Port=2
  Vc : Outport  Port=3
  wires:
  In1/1 -> Va/1, Product1/2, Product2/2
  In2/1 -> Product/1, Product3/2
  Add/1 -> Vb/1
  Product3/1 -> Add1/2
  Constant/1 -> Product1/1
  Constant2/1 -> Product2/1
  Product/1 -> Add/2
  Constant1/1 -> Product/2
  Product1/1 -> Add/1
  Product2/1 -> Add1/1
  Add1/1 -> Vc/1
  Constant3/1 -> Product3/1

== system FOC_physical_2/SVPWM/Subsystem ==
  Valpha : Inport
  Vbeta : Inport  Port=2
  Atan2 : Trigonometry  Operator=atan2
  Display : Display
  Display1 : Display
  Math Function : Math  Operator=square
  Math Function1 : Math  Operator=square
  Scope : Scope
  Sqrt1 : Sqrt
  Sum : Sum  Inputs=|++
  Vref : Outport
  angle : Outport  Port=2
  wires:
  Math Function1/1 -> Sum/2
  Valpha/1 -> Atan2/2, Math Function/1
  Vbeta/1 -> Atan2/1, Math Function1/1
  Sqrt1/1 -> Display/1, Vref/1, Scope/1
  Math Function/1 -> Sum/1
  Atan2/1 -> angle/1, Display1/1
  Sum/1 -> Sqrt1/1

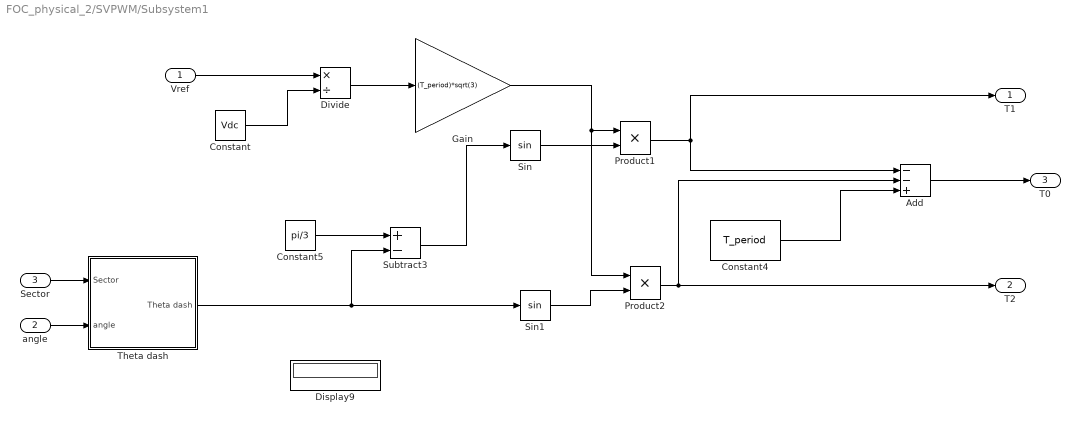
== system FOC_physical_2/SVPWM/Subsystem1 ==
  Vref : Inport
  angle : Inport  Port=2
  Sector : Inport  Port=3
  Add : Sum  Inputs=--+
  Constant : Constant  Value=Vdc
  Constant4 : Constant  Value=T_period
  Constant5 : Constant  Value=pi/3
  Display9 : Display
  Divide : Product  Inputs=*/
  Gain : Gain  Gain=(T_period)*sqrt(3)
  Product1 : Product
  Product2 : Product
  Sin : Trigonometry
  Sin1 : Trigonometry
  Subtract3 : Sum  Inputs=+-
  Theta dash : Subsystem
  T1 : Outport
  T2 : Outport  Port=2
  T0 : Outport  Port=3
  wires:
  Sector/1 -> Theta dash/1(Sector)
  Constant5/1 -> Subtract3/1
  angle/1 -> Theta dash/2(angle)
  Divide/1 -> Gain/1
  Vref/1 -> Divide/1
  Constant/1 -> Divide/2
  Subtract3/1 -> Sin/1
  Gain/1 -> Product2/1, Product1/1
  Sin/1 -> Product1/2
  Sin1/1 -> Product2/2
  Product1/1 -> T1/1, Add/1
  Constant4/1 -> Add/3
  Product2/1 -> Add/2, T2/1
  Add/1 -> T0/1
  Theta dash/1(Theta dash) -> Sin1/1, Subtract3/2

== system FOC_physical_2/SVPWM/Subsystem2 ==
  T1 : Inport
  T2 : Inport  Port=2
  T0 : Inport  Port=3
  Sector definiton : Inport  Port=4
  Display : Display
  Fcn : Fcn  Expr=(T_period)-(u(3)/2)
  Fcn1 : Fcn  Expr=u(2)+(u(3)/2)
  Fcn2 : Fcn  Expr=u(3)/2
  Fcn3 : Fcn  Expr=u(1)+(u(3)/2)
  MATLAB Function : MATLAB Function  TreatAsAtomicUnit=on
  Mux : Mux  Inputs=3
  TS1 : Outport
  TS3 : Outport  Port=2
  TS5 : Outport  Port=3
  wires:
  MATLAB Function/1(TS1) -> TS1/1
  MATLAB Function/3(TS5) -> TS5/1
  MATLAB Function/2(TS3) -> TS3/1
  T1/1 -> Mux/1
  T2/1 -> Mux/2
  T0/1 -> Mux/3
  Mux/1 -> Display/1, Fcn1/1, Fcn/1, Fcn3/1, Fcn2/1
  Fcn/1 -> MATLAB Function/1(u)
  Fcn1/1 -> MATLAB Function/2(v)
  Fcn2/1 -> MATLAB Function/3(w)
  Fcn3/1 -> MATLAB Function/4(g)
  Sector definiton/1 -> MATLAB Function/5(S)

== system FOC_physical_2/SVPWM/Subsystem3 ==
  TS1 : Inport
  TS3 : Inport  Port=2
  TS5 : Inport  Port=3
  Carrier : Inport  Port=4
  Relational Operator : RelationalOperator  OutDataTypeStr=boolean  RndMeth=Simplest  InputSameDT=off
  Relational Operator1 : RelationalOperator  OutDataTypeStr=boolean  RndMeth=Simplest  InputSameDT=off
  Relational Operator2 : RelationalOperator  OutDataTypeStr=boolean  RndMeth=Simplest  InputSameDT=off
  Scope : Scope  NumInputPorts=3
  Pwm1 : Outport
  PWM3 : Outport  Port=2
  PWM5 : Outport  Port=3
  wires:
  TS1/1 -> Scope/1, Relational Operator/1
  TS3/1 -> Relational Operator1/1
  TS5/1 -> Relational Operator2/1
  Carrier/1 -> Scope/2, Relational Operator/2, Relational Operator1/2, Relational Operator2/2
  Relational Operator/1 -> Scope/3, Pwm1/1
  Relational Operator1/1 -> PWM3/1
  Relational Operator2/1 -> PWM5/1

== system FOC_physical_2/SVPWM/Subsystem4 ==
  TS1 : Inport
  TS3 : Inport  Port=2
  TS5 : Inport  Port=3
  NOT : Logic  Operator=NOT  IconShape=distinctive  AllPortsSameDT=off  OutDataTypeStr=boolean
  NOT1 : Logic  Operator=NOT  IconShape=distinctive  AllPortsSameDT=off  OutDataTypeStr=boolean
  NOT2 : Logic  Operator=NOT  IconShape=distinctive  AllPortsSameDT=off  OutDataTypeStr=boolean
  S1 : Outport
  S2 : Outport  Port=2
  S3 : Outport  Port=3
  S4 : Outport  Port=4
  S5 : Outport  Port=5
  S6 : Outport  Port=6
  wires:
  NOT2/1 -> S2/1
  TS5/1 -> NOT2/1, S5/1
  NOT1/1 -> S6/1
  TS3/1 -> S3/1, NOT1/1
  NOT/1 -> S4/1
  TS1/1 -> S1/1, NOT/1

== system FOC_physical_2/SVPWM/Valpha and Vbeta Clark Trans ==
  Va : Inport
  Vb : Inport  Port=2
  Vc : Inport  Port=3
  Add : Sum  Inputs=+++
  Add1 : Sum  Inputs=+-
  Gain : Gain  Gain=2/3
  Gain1 : Gain  Gain=-1/2
  Gain2 : Gain  Gain=-1/2
  Gain3 : Gain  Gain=2/3
  Gain5 : Gain  Gain=sqrt(3)/2
  Valpha : Outport
  Vbeta : Outport  Port=2
  wires:
  Gain1/1 -> Add/2
  Va/1 -> Add/1
  Add1/1 -> Gain5/1
  Gain2/1 -> Add/3
  Add/1 -> Gain/1
  Gain/1 -> Valpha/1
  Gain3/1 -> Vbeta/1
  Vb/1 -> Add1/1, Gain1/1
  Vc/1 -> Add1/2, Gain2/1
  Gain5/1 -> Gain3/1

== system FOC_physical_2/SVPWM Technique/Gate Signals ==
  PWM1 : Inport
  PWM3 : Inport  Port=2
  PWM5 : Inport  Port=3
  NOT : Logic  Operator=NOT  IconShape=distinctive  AllPortsSameDT=off  OutDataTypeStr=boolean
  NOT1 : Logic  Operator=NOT  IconShape=distinctive  AllPortsSameDT=off  OutDataTypeStr=boolean
  NOT2 : Logic  Operator=NOT  IconShape=distinctive  AllPortsSameDT=off  OutDataTypeStr=boolean
  T1 : Outport
  T2 : Outport  Port=2
  T3 : Outport  Port=3
  T4 : Outport  Port=4
  T5 : Outport  Port=5
  T6 : Outport  Port=6
  wires:
  NOT2/1 -> T2/1
  PWM5/1 -> NOT2/1, T5/1
  PWM3/1 -> NOT1/1, T3/1
  NOT1/1 -> T6/1
  NOT/1 -> T4/1
  PWM1/1 -> NOT/1, T1/1

== system FOC_physical_2/SVPWM Technique/PWM ==
  Ts1 : Inport
  Ts3 : Inport  Port=2
  Ts5 : Inport  Port=3
  Carrier : Inport  Port=4
  Mux : Mux  Inputs=2
  Relational Operator : RelationalOperator  OutDataTypeStr=boolean  RndMeth=Simplest  InputSameDT=off
  Relational Operator1 : RelationalOperator  OutDataTypeStr=boolean  RndMeth=Simplest  InputSameDT=off
  Relational Operator2 : RelationalOperator  OutDataTypeStr=boolean  RndMeth=Simplest  InputSameDT=off
  Scope : Scope  NumInputPorts=2
  PWM1 : Outport
  PWM3 : Outport  Port=2
  PWM5 : Outport  Port=3
  wires:
  Mux/1 -> Scope/1
  Relational Operator2/1 -> PWM5/1
  Relational Operator1/1 -> PWM3/1
  Relational Operator/1 -> PWM1/1, Scope/2
  Carrier/1 -> Relational Operator/2, Mux/2, Relational Operator1/2, Relational Operator2/2
  Ts5/1 -> Relational Operator2/1
  Ts3/1 -> Relational Operator1/1
  Ts1/1 -> Relational Operator/1, Mux/1

== system FOC_physical_2/SVPWM Technique/Step 1- Determine Vd, Vq, Vref, and angle ==
  Va* : Inport
  Vb* : Inport  Port=2
  Vc* : Inport  Port=3
  Polar form : Subsystem
  "Power variant Clark transformation " : Subsystem
  Scope : Scope  NumInputPorts=2
  V ref : Outport
  angle : Outport  Port=2
  wires:
  Vc*/1 -> "Power variant Clark transformation "/3(Vc)
  Vb*/1 -> "Power variant Clark transformation "/2(Vb)
  Va*/1 -> "Power variant Clark transformation "/1(Va)
  Polar form/2(angle) -> angle/1
  Polar form/1(V ref) -> V ref/1
  "Power variant Clark transformation "/2(V beta) -> Polar form/2(In2), Scope/2
  "Power variant Clark transformation "/1(V alpha) -> Polar form/1(In1), Scope/1

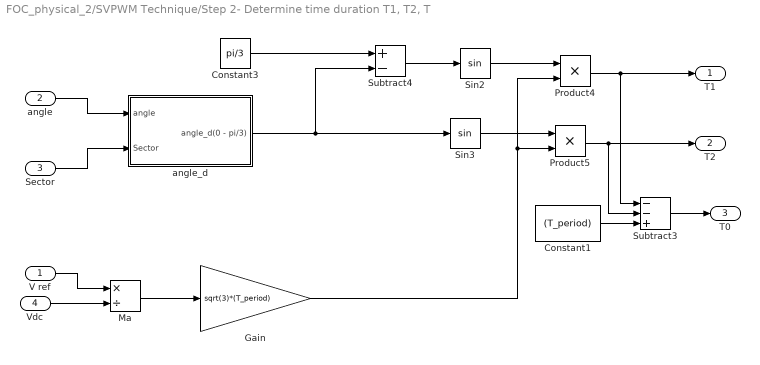
== system FOC_physical_2/SVPWM Technique/Step 2- Determine time duration T1, T2, T ==
  V ref : Inport
  angle : Inport  Port=2
  Sector : Inport  Port=3
  Vdc : Inport  Port=4
  Constant1 : Constant  Value=(T_period)
  Constant3 : Constant  Value=pi/3
  Gain : Gain  Gain=sqrt(3)*(T_period)
  Ma : Product  Inputs=*/
  Product4 : Product
  Product5 : Product
  Sin2 : Trigonometry
  Sin3 : Trigonometry
  Subtract3 : Sum  Inputs=--+
  Subtract4 : Sum  Inputs=+-
  angle_d : Subsystem
  T1 : Outport
  T2 : Outport  Port=2
  T0 : Outport  Port=3
  wires:
  angle_d/1(angle_d(0 - pi/3)) -> Subtract4/2, Sin3/1
  Constant1/1 -> Subtract3/3
  Subtract3/1 -> T0/1
  Product5/1 -> T2/1, Subtract3/2
  Sin3/1 -> Product5/1
  Product4/1 -> T1/1, Subtract3/1
  Gain/1 -> Product5/2, Product4/2
  Sin2/1 -> Product4/1
  Ma/1 -> Gain/1
  Subtract4/1 -> Sin2/1
  Constant3/1 -> Subtract4/1
  Vdc/1 -> Ma/2
  V ref/1 -> Ma/1
  Sector/1 -> angle_d/2(Sector)
  angle/1 -> angle_d/1(angle)

== system FOC_physical_2/SVPWM Technique/Step 3- Determine the switching time of each transistor (S1 to S6)  ==
  T1 : Inport
  T2 : Inport  Port=2
  T0 : Inport  Port=3
  S : Inport  Port=4
  Fcn : Fcn  Expr=(T_period)-u(3)/2
  Fcn1 : Fcn  Expr=u(3)/2+u(2)
  Fcn2 : Fcn  Expr=u(3)/2
  Fcn3 : Fcn  Expr=u(3)/2+u(1)
  Mux1 : Mux  Inputs=3
  Sector detection1 : MATLAB Function  TreatAsAtomicUnit=on
  Ts1 : Outport
  Ts3 : Outport  Port=2
  Ts5 : Outport  Port=3
  wires:
  Sector detection1/1(Ts1) -> Ts1/1
  Sector detection1/3(Ts5) -> Ts5/1
  Sector detection1/2(Ts3) -> Ts3/1
  T0/1 -> Mux1/3
  T2/1 -> Mux1/2
  T1/1 -> Mux1/1
  Fcn2/1 -> Sector detection1/4(w)
  Fcn/1 -> Sector detection1/2(u)
  Fcn3/1 -> Sector detection1/5(g)
  Mux1/1 -> Fcn2/1, Fcn3/1, Fcn1/1, Fcn/1
  Fcn1/1 -> Sector detection1/3(v)
  S/1 -> Sector detection1/1(s)

== system FOC_physical_2/Voltage limits/If Action Subsystem ==
  In3 : Inport
  In4 : Inport  Port=2
  Action Port : ActionPort  ActionPortLabel=if(u1 <= 0)
  Cast To Single : DataTypeConversion  OutDataTypeStr=single  SaturateOnIntegerOverflow=off  RndMeth=Floor
  Cast To Single1 : DataTypeConversion  OutDataTypeStr=single  SaturateOnIntegerOverflow=off  RndMeth=Floor
  Out2 : Outport
  Out3 : Outport  Port=2
  wires:
  In3/1 -> Cast To Single/1
  In4/1 -> Cast To Single1/1
  Cast To Single/1 -> Out2/1
  Cast To Single1/1 -> Out3/1

== system FOC_physical_2/Voltage limits/If Action Subsystem1 ==
  In3 : Inport
  In4 : Inport  Port=2
  Action Port : ActionPort  ActionPortLabel=else
  Divide1 : Product  Inputs=*/  OutDataTypeStr=single
  Divide2 : Product  Inputs=/*  OutDataTypeStr=single
  Gain : Gain  Gain=sqrt(3)
  Gain1 : Gain  Gain=325 * .95
  Gain2 : Gain  Gain=325 * .95
  Square : Math  Operator=square  OutDataTypeStr=single
  Square Root : Sqrt  OutDataTypeStr=single  IntermediateResultsDataTypeStr=single
  Square1 : Math  Operator=square  OutDataTypeStr=single
  Sum : Sum  OutDataTypeStr=single  AccumDataTypeStr=single
  Out2 : Outport
  Out3 : Outport  Port=2
  wires:
  Divide1/1 -> Out2/1
  Divide2/1 -> Out3/1
  Square/1 -> Sum/1
  In3/1 -> Gain1/1, Square/1
  Sum/1 -> Square Root/1
  Gain2/1 -> Divide2/2
  Gain/1 -> Divide2/1, Divide1/2
  Gain1/1 -> Divide1/1
  Square1/1 -> Sum/2
  Square Root/1 -> Gain/1
  In4/1 -> Square1/1, Gain2/1

== system FOC_physical_2/voltage limits by maintaining the same ration/Normal_Voltage ==
  Vq_ref_new : Inport
  Vd_ref_new : Inport  Port=2
  Action Port : ActionPort  ActionPortLabel=if(u1 <= 0)
  Data Type Conversion : DataTypeConversion  OutDataTypeStr=single  SaturateOnIntegerOverflow=off  RndMeth=Floor
  Data Type Conversion1 : DataTypeConversion  OutDataTypeStr=single  SaturateOnIntegerOverflow=off  RndMeth=Floor
  Vq_ref_1 : Outport
  Vd_ref_1 : Outport  Port=2
  wires:
  Vq_ref_new/1 -> Data Type Conversion/1
  Vd_ref_new/1 -> Data Type Conversion1/1
  Data Type Conversion/1 -> Vq_ref_1/1
  Data Type Conversion1/1 -> Vd_ref_1/1

== system FOC_physical_2/voltage limits by maintaining the same ration/Voltage_to_be_Limited ==
  Vq_ref_new : Inport
  Vd_ref_new : Inport  Port=2
  Action Port : ActionPort  ActionPortLabel=else
  Divide1 : Product  Inputs=*/  OutDataTypeStr=single
  Divide2 : Product  Inputs=/*  OutDataTypeStr=single
  Gain : Gain  Gain=sqrt(3)
  Gain1 : Gain  Gain=Vdc * ma
  Gain2 : Gain  Gain=Vdc * ma
  Square : Math  Operator=square  OutDataTypeStr=single
  Square Root : Sqrt  OutDataTypeStr=single  IntermediateResultsDataTypeStr=single
  Square1 : Math  Operator=square  OutDataTypeStr=single
  Sum : Sum  OutDataTypeStr=single  AccumDataTypeStr=single
  Vq_ref_2 : Outport
  Vd_ref_2 : Outport  Port=2
  wires:
  Vq_ref_new/1 -> Gain1/1, Square/1
  Sum/1 -> Square Root/1
  Vd_ref_new/1 -> Square1/1, Gain2/1
  Square1/1 -> Sum/2
  Square/1 -> Sum/1
  Divide1/1 -> Vq_ref_2/1
  Square Root/1 -> Gain/1
  Divide2/1 -> Vd_ref_2/1
  Gain/1 -> Divide2/1, Divide1/2
  Gain1/1 -> Divide1/1
  Gain2/1 -> Divide2/2

== system FOC_physical_2/SVPWM/Subsystem1/Theta dash ==
  Sector : Inport
  angle : Inport  Port=2
  Constant : Constant
  Display : Display
  Gain : Gain  Gain=(pi/3)
  Subtract : Sum  Inputs=-+
  Subtract1 : Sum  Inputs=-+
  Theta dash : Outport
  wires:
  angle/1 -> Subtract/2
  Gain/1 -> Subtract/1
  Constant/1 -> Subtract1/1
  Sector/1 -> Subtract1/2
  Subtract1/1 -> Gain/1
  Subtract/1 -> Display/1, Theta dash/1

== system FOC_physical_2/SVPWM Technique/Step 1- Determine Vd, Vq, Vref, and angle/Polar form ==
  In1 : Inport
  In2 : Inport  Port=2
  Add : Sum
  Atan2 : Trigonometry  Operator=atan2
  Sqrt : Sqrt
  Square : Math  Operator=square
  Square1 : Math  Operator=square
  V ref : Outport
  angle : Outport  Port=2
  wires:
  In1/1 -> Square/1, Atan2/2
  Add/1 -> Sqrt/1
  Sqrt/1 -> V ref/1
  In2/1 -> Square1/1, Atan2/1
  Atan2/1 -> angle/1
  Square/1 -> Add/1
  Square1/1 -> Add/2

== system FOC_physical_2/SVPWM Technique/Step 1- Determine Vd, Vq, Vref, and angle/Power variant Clark transformation  ==
  Va : Inport
  Vb : Inport  Port=2
  Vc : Inport  Port=3
  Gain : Gain  Gain=0.5
  Gain1 : Gain  Gain=0.5
  Gain2 : Gain  Gain=2/3
  Gain3 : Gain  Gain=sqrt(3)/2
  Gain4 : Gain  Gain=2/3
  Sum : Sum  Inputs=+--
  Sum1 : Sum  Inputs=+-
  V alpha : Outport
  V beta : Outport  Port=2
  wires:
  Gain4/1 -> V beta/1
  Gain2/1 -> V alpha/1
  Vb/1 -> Gain/1, Sum1/1
  Gain/1 -> Sum/2
  Sum1/1 -> Gain3/1
  Gain1/1 -> Sum/3
  Vc/1 -> Gain1/1, Sum1/2
  Sum/1 -> Gain2/1
  Gain3/1 -> Gain4/1
  Va/1 -> Sum/1

== system FOC_physical_2/SVPWM Technique/Step 2- Determine time duration T1, T2, T/angle_d ==
  angle : Inport
  Sector : Inport  Port=2
  Constant3 : Constant
  Gain : Gain  Gain=pi/3
  Subtract4 : Sum  Inputs=-+
  Subtract5 : Sum  Inputs=+-
  angle_d(0 - pi/3) : Outport
  wires:
  Gain/1 -> Subtract4/1
  Subtract5/1 -> Gain/1
  Constant3/1 -> Subtract5/2
  Subtract4/1 -> angle_d(0 - pi/3)/1
  Sector/1 -> Subtract5/1
  angle/1 -> Subtract4/2

== matlab function FOC_physical_2/SVPWM/Subsystem2/MATLAB Function ==
  data: TS1 output; u input; TS3 output; TS5 output; v input; w input; g input; S input
function [TS1, TS3,TS5] = fcn(u, v, w, g,S)

switch S
    case 1
        TS1 = u;
        TS3 = v;
        TS5 = w;
    case 2
        TS1 = g;
        TS3 = u;
        TS5 = w;
    case 3
        TS1 = w;
        TS3 = u;
        TS5 = v;
    case 4
        TS1 = w;
        TS3 = g;
        TS5 = u;
    case 5
        TS1 = v;
        TS3 = w;
        TS5 = u;
    case 6
        TS1 = u;
        TS3 = w;
        TS5 = g;
    otherwise
      TS1=0;  
      TS3=0;  
      TS5=0; 
end
end
